simulink model "ATOM_simple_planning_simulator"  (R2026a)
settings: Solver=ode4  StopTime=100  FixedStep=0.01
StopFcn:
  | % Put every new figure in the same MATLAB Figures window as a docked tab.
  | set(groot, 'defaultFigureWindowStyle', 'docked');
  | 
  | if exist('costmap_active', 'var') && ...
  |     exist('vehicle', 'var') && ...
  |     exist('parking_path', 'var') && ...
  |     ~isempty(parking_path)
  | 
  |      plotPlan(costmap_active, vehicle, parking_path);
  | 
  |  else
  | 
  |      warning('No valid parking path is available for plotting.');
  | 
  |  end
  | 
  |  PlotControllerReferences( ...
  |      out.controller_reference_log);
  | 
  |  PlotControllerTracking( ...
  |      out.controller_tracking_log);
  | 
model workspace (MAT data in the model file):
  vehicle : object (value not decoded)
symbols that are objects in the model workspace (value not decoded): vehicle
undefined symbols (not defined in the file): delta_f_LUT, gain4WS_LUT, k_ref_LUT, kappa_gain_BP, Ki, Kp, lateral, longitudinal, planning_validator, rr_gain_BP, rr_LUT, stanley, velocity_smoother
libraries: slpidlib x1
(part 8 of 8)

== matlab function ATOM_simple_planning_simulator/Vehicle_Model2/Vehicle Dynamics/MATLAB Function ==
  data: state input Bus: VehicleInternalStateBus size=1; d_state output Bus: VehicleInternalStateBus size=1; command input Bus: ControlCMDBus size=1; veh input; rear_steering_command input
function d_state = vehicleDynamics(state, command, veh, rear_steering_command)

%%%%%%%%%%%%%%%%%%%%%%%%%%%%%%%%%%%%%%
%%%%%%%%%%%%%%%%%%%%%%%%%%%%%%%%%%%%%%
% Description:
% This vehicleDynamics model follows DELAY_STEER_ACC_GEARED
% model, it doesn't presents a model for gear management
% since its not something we're going to modify on Autoware for 4WS
% implementation.
%
% Inputs:
% - state: VehicleInternalStateBus. It contains the state of the vehicle
%          at time instant t. 
% - command: /control/command/control_cmd topic --> ControlCMDBus.
%          It contains the desired acc and steering commands coming from
%          the control region.
%
% - Parameters
% - vehicle: vehicle parameters struct defined in vehicleParameters.m.

% Outputs: 
% - d_state: It contains the derivative of the state of the vehicle at time
%          instant t+1.
%%%%%%%%%%%%%%%%%%%%%%%%%%%%%%%%%%%%%%
%%%%%%%%%%%%%%%%%%%%%%%%%%%%%%%%%%%%%%


% inside MATLAB Function: input is veh_in (1xN double)
v = veh; % 1xN numeric row

vehicle.param.wheel_radius    = v(1);
vehicle.param.wheel_width     = v(2);
vehicle.param.wheel_base      = v(3);
vehicle.param.wheel_tread     = v(4);
vehicle.param.front_overhang  = v(5);
vehicle.param.rear_overhang   = v(6);
vehicle.param.left_overhang   = v(7);
vehicle.param.right_overhang  = v(8);
vehicle.param.vehicle_height  = v(9);
vehicle.param.max_steer_angle = v(10);

% decode integer-coded enums (example)
vehicle.sim.vehicle_model_type = int32(v(11));    % or map to strings if needed
vehicle.sim.initialize_source  = int32(v(12));

vehicle.sim.timer_sampling_time_ms = v(13);
vehicle.sim.add_measurement_noise = logical(v(14));
vehicle.sim.vel_lim        = v(15);
vehicle.sim.vel_rate_lim   = v(16);
vehicle.sim.steer_lim      = v(17);
vehicle.sim.steer_rate_lim = v(18);
vehicle.sim.acc_time_delay = v(19);
vehicle.sim.acc_time_constant = v(20);
vehicle.sim.steer_time_delay   = v(21);
vehicle.sim.steer_time_constant= v(22);
vehicle.sim.x_stddev = v(23);
vehicle.sim.y_stddev = v(24);
vehicle.sim.steer_dead_band = v(25);
vehicle.sim.steer_bias = v(26);
vehicle.sim.debug_acc_scaling_factor = v(27);
vehicle.sim.debug_steer_scaling_factor = v(28);

% Parameter for 4WS
vehicle.param.rear_steering_ratio = veh(29);
rear_steering_ratio = vehicle.param.rear_steering_ratio;

%% ==========================
% Saturation function
% ===========================

sat = @(val, upper, lower) min(max(val,lower),upper);



%% ==========================
% Current state
% ===========================

vx = sat( ...
    state.vx,...
    vehicle.sim.vel_lim,...
   -vehicle.sim.vel_lim);


acc = sat( ...
    state.acc,...
    vehicle.sim.vel_rate_lim,...
   -vehicle.sim.vel_rate_lim);


yaw = state.yaw;

steer_front = state.steer_front;
steer_rear = state.steer_rear;          % Modified for 4WS  


%% ==========================
% Input commands
% ===========================

acc_des = sat( ...
    command.longitudinal.acceleration,...
    vehicle.sim.vel_rate_lim,...
   -vehicle.sim.vel_rate_lim);


acc_des = acc_des * ...
    vehicle.sim.debug_acc_scaling_factor;



steer_front_des = sat( ...
    command.lateral.steering_tire_angle,...
    vehicle.sim.steer_lim,...
   -vehicle.sim.steer_lim);


steer_front_des = steer_front_des * ...
    vehicle.sim.debug_steer_scaling_factor;

steer_rear_des = sat( ...                                            % Modified for 4WS
    rear_steering_command,...
    vehicle.sim.steer_lim,...
    -vehicle.sim.steer_lim);


steer_rear_des = steer_rear_des * ...                                % Modified for 4WS
    vehicle.sim.debug_steer_scaling_factor;



%% ==========================
% Steering dynamics
% ===========================

% getSteer() in simple_planning_simulator corresponds to state.steer
% From the phisical vehicle front_steer and rear_steer are measured.

steer_diff_front = steer_front - steer_front_des;

steer_diff_rear = steer_rear  - steer_rear_des;             % Modified for 4WS


% dead band

if steer_diff_front > vehicle.sim.steer_dead_band

    steer_diff_with_dead_band_front = ...
        steer_diff_front - vehicle.sim.steer_dead_band;


elseif steer_diff_front < -vehicle.sim.steer_dead_band

    steer_diff_with_dead_band_front = ...
        steer_diff_front + vehicle.sim.steer_dead_band;


else

    steer_diff_with_dead_band_front = 0;

end



if steer_diff_rear > vehicle.sim.steer_dead_band            % Modified for 4WS

    steer_diff_with_dead_band_rear = ...
        steer_diff_rear - vehicle.sim.steer_dead_band;


elseif steer_diff_rear < -vehicle.sim.steer_dead_band

    steer_diff_with_dead_band_rear = ...
        steer_diff_rear + vehicle.sim.steer_dead_band;


else

    steer_diff_with_dead_band_rear = 0;

end



steer_rate_front = sat( ...
    -steer_diff_with_dead_band_front / vehicle.sim.steer_time_constant,...
     vehicle.sim.steer_rate_lim,...
    -vehicle.sim.steer_rate_lim);

steer_rate_rear = sat( ...                                                  % Modified for 4WS
    -steer_diff_with_dead_band_rear / vehicle.sim.steer_time_constant,...
    vehicle.sim.steer_rate_lim,...
    -vehicle.sim.steer_rate_lim);



%% ==========================
% State derivative
% ===========================

%--------------------------------------------------------------
% 4WS kinematic bicycle model
%
% Assumptions:
%   - Pure rolling
%   - alpha_f = alpha_r = 0
%   - No tire dynamics
%   - No lateral slip dynamics
%
% beta is the geometric vehicle sideslip angle. Since Autoware defines
% reference frame of the vehicle equal to centre of the rear axle, then
% beta = steer_rear
%--------------------------------------------------------------

L = vehicle.param.wheel_base;


beta = steer_rear;                              % Modified for 4WS


vel = vx/cos(beta);                             % Modified for 4WS


yaw_rate = ...                                  % Modified for 4WS
    (vx/L) * ...
    (tan(steer_front)-tan(steer_rear));


d_state.x = vel*cos(yaw + beta);                % Modified for 4WS

d_state.y = vel*sin(yaw + beta);                % Modified for 4WS


d_state.yaw = yaw_rate;                         % Modified for 4WS


d_state.vx = acc + yaw_rate*vel*sin(beta);


d_state.steer_front = steer_rate_front;

d_state.steer_rear = steer_rate_rear;           % Modified for 4WS

d_state.acc = ...
    -(acc-acc_des)/vehicle.sim.acc_time_constant;

end

== matlab function ATOM_simple_planning_simulator/Vehicle_Model2/localization//acceleration function ==
  data: state input Bus: VehicleInternalStateBus; accel output Bus: AccelerationBus; veh input
function accel = IntStateToAccelerationState(state,veh)

L = veh(3);

vx = state.vx;
ax = state.acc;

delta_f = state.steer_front;
delta_r = state.steer_rear;

yaw_rate = (vx/L)*(tan(delta_f)-tan(delta_r));

ay = vx*yaw_rate;

accel.acceleration.linear.x = ax;
accel.acceleration.linear.y = ay;
accel.acceleration.linear.z = 0;

accel.acceleration.angular.x = 0;
accel.acceleration.angular.y = 0;
accel.acceleration.angular.z = 0;

end
